simulink model "simulink_example"  (R2024b)
settings: Solver=VariableStepAuto  StartTime=0.0  StopTime=10.0  RelTol=1e-3
settings Model: Creator=33657  LastModifiedBy=33657

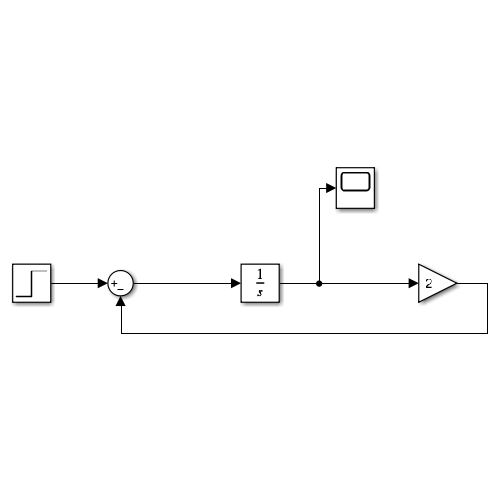
[thumbnail: Simulink's stored preview of the top-level diagram]
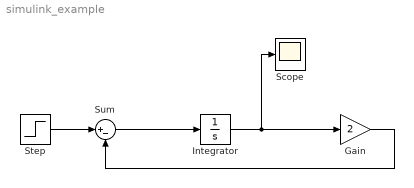
== system simulink_example ==
  Gain : Gain  Gain=2
  Integrator : Integrator
  Scope : Scope
  Step : Step  SampleTime=0
  Sum : Sum  Inputs=|+-
  wires:
  Step/1 -> Sum/1
  Sum/1 -> Integrator/1
  Integrator/1 -> Scope/1, Gain/1
  Gain/1 -> Sum/2
